simulink model "flightControlSystem"  (R2026b)
settings: Solver=ode3  StopTime=TFinal
PreLoadFcn:
  | InitVars;
undefined symbols (not defined in the file): control_power, feedforward_gains, integrator_limits, MC_PITCH_P, MC_PITCHRATE_D, MC_PITCHRATE_I, MC_PITCHRATE_MAX, MC_PITCHRATE_P, MC_ROLL_P, MC_ROLLRATE_D, MC_ROLLRATE_I, MC_ROLLRATE_MAX, MC_ROLLRATE_P, MC_YAW_P, MC_YAW_TQ_CUTOFF, MC_YAW_WEIGHT, MC_YAWRATE_D, MC_YAWRATE_I, MC_YAWRATE_MAX, MC_YAWRATE_P, MPC_ACC_DECOUPLE, MPC_LAND_ALT1, MPC_LAND_ALT2, MPC_LAND_ALT3, MPC_LAND_CRWL, MPC_LAND_SPEED, MPC_THR_HOVER, MPC_THR_MAX, MPC_THR_MIN, MPC_THR_XY_MARG, MPC_TILTMAX_AIR, MPC_VELD_LP, MPC_XY_P, MPC_XY_VEL_D_ACC, MPC_XY_VEL_I_ACC, MPC_XY_VEL_MAX, MPC_XY_VEL_P_ACC, MPC_Z_P, MPC_Z_VEL_D_ACC, MPC_Z_VEL_I_ACC, MPC_Z_VEL_MAX_DN, MPC_Z_VEL_MAX_UP, MPC_Z_VEL_P_ACC, SampleTime, timestamp
libraries: px4uORBlib x9, vrlib x8, aerolibutil x8, simulink x4, px4Utilslib x4, sharedutil x3, matrix_library x3, raspberrypiutilitieslib x2, px4Peripheralslib x2, sharedtransform x1, px4Sensorslib x1
(part 1 of 4)
settings Model: SimulationMode=external  Creator=The MathWorks, Inc.  LastModifiedBy=merwyn
settings SolverCC: AutoInsertRateTranBlk=on  PositivePriorityOrder=on
settings OptimizationCC: DifferentSizesBufferReuse=on  EfficientTunableParamExpr=on  EnhancedBackFolding=on  MaxStackSize=64  OptimizationCustomize=off  OptimizeBlockOrder=speed  PassReuseOutputArgsAs=Individual arguments  RemoveInternalMemoryZeroInit=on  RemoveRootLevelIOMemoryZeroInit=on
settings DebuggingCC: ParameterPrecisionLossMsg=none  ParameterTunabilityLossMsg=error
settings HardwareCC: ProdHWDeviceType=ARM Compatible->ARM Cortex  ProdLargestAtomicFloat=Double  ProdLargestAtomicInteger=Long  ProdLongLongMode=on
settings SFSimCC: MATLABDynamicMemAlloc=off  SimTargetLang=C++
settings RTWCC: Description=Embedded Coder  GenCodeOnly=on  HardwareBoard=PX4 Pixhawk 6c  SystemTargetFile=ert.tlc  TLCOptions="-aInlineSetEventsForThisBaseRateFcn=TLC_FALSE -aSuppressMultiTaskScheduler=TLC_FALSE  -aRateBasedStepFcn=0"  TargetLang=C++  TemplateMakefile=ert_default_tmf  Toolchain=GNU Tools for PX4 Autopilots
settings CodeAppCC: ForceParamTrailComments=on  IgnoreCustomStorageClasses=off  InsertBlockDesc=on  OperatorAnnotations=on  SFDataObjDesc=on  SimulinkDataObjDesc=on
settings ERTTargetCC: ExtModeIntrfLevel=Level2 - Open  ExtModeMexFile=ext_xcp  ExtModeStaticAlloc=on  SupportContinuousTime=on  SupportVariableSizeSignals=on

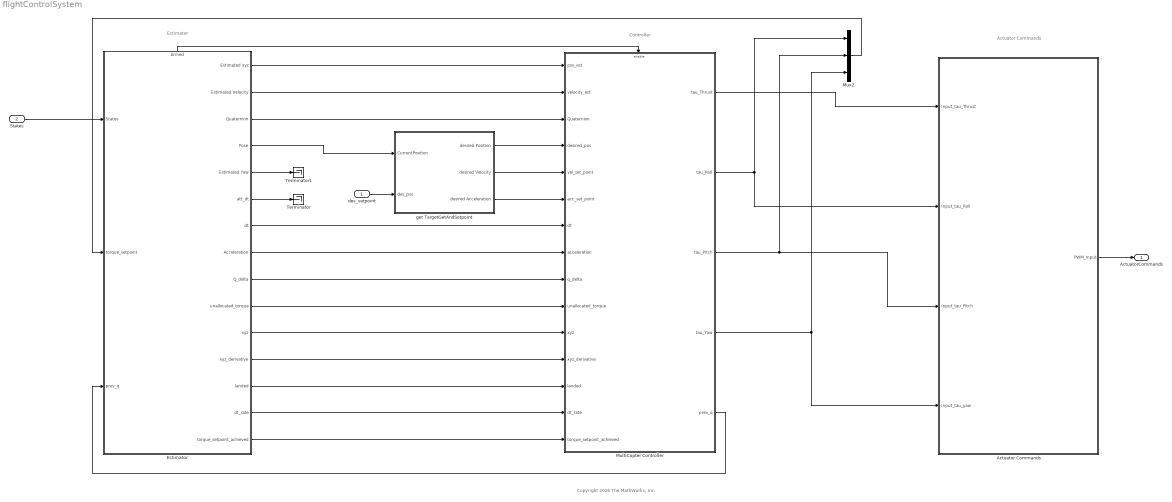
== system flightControlSystem ==
  note: Actuator Commands
  note: Estimator
  note: Controller
  note: Copyright 2026 The MathWorks, Inc.
  des_setpoint : Inport  OutDataTypeStr=Bus: desiredTargetSetpoints
  States : Inport  Port=2  OutDataTypeStr=Bus: UAVStatesBus
  Actuator Commands : Subsystem  Variant=on
  Estimator : Subsystem  Variant=on
      settings: PortSchema="{\"entries\":[{\"content\":{\"sides\":[{\"content\":{\"connectorIds\":[\"In1\",\"In2\",\"In3\"]},\"type\":\"ConnectorPlacement.EquallySpacedRectSide\",\"uuid\":\"982d90d8-ff1f-4cb9-8e33-8baf717922ad\"},{\"content\":{\"connectorIds\":[\"Out1\",\"Out2\",\"Out3\",\"Out4\",\"Out5\",\"Out6\",\"Out7\",\"Out8\",\"Out9\",\"Out10\",\"Out11\",\"Out12\",\"Out13\",\"Out14\",\"Out15\"],\"side\":\"RIGHT\"},\"type\":\"ConnectorPlacement.EquallySpacedRectSide\",\"uuid\":\"20bc02a1-8188-433b-a626-e8822f00966c\"},{\"content\":{\"connectorIds\":[\"Out16\"],\"side\":\"TOP\"},\"type\":\"ConnectorPlacement.EquallySpacedRectSide\",\"uuid\":\"edaeaf83-210e-410d-8d39-7cda3629118d\"}]},\"type\":\"ConnectorPlacement.EquallySpacedConnector\",\"uuid\":\"c0d6638f-6096-4882-ba89-b56950bc4adf\"}],\"packageUris\":[\"http://schema.mathworks.com/mf0/Connector/R2020b\"],\"version\":\"1.0\"}"
  MultiCopter Controller : Subsystem
  Mux2 : Mux  Inputs=3
  Terminator : Terminator
  Terminator1 : Terminator
  get TargetGetAndSetpoint : Subsystem  Variant=on
  ActuatorCommands : Outport  OutDataTypeStr=Bus: setPWMInput
  wires:
  MultiCopter Controller/2(tau_Roll) -> Actuator Commands/2(Input_tau_Roll), Mux2/1
  MultiCopter Controller/1(tau_Thrust) -> Actuator Commands/1(Input_tau_Thrust)
  Estimator/11(xyz) -> MultiCopter Controller/11(xyz)
  MultiCopter Controller/4(tau_Yaw) -> Mux2/3, Actuator Commands/4(Input_tau_yaw)
  Estimator/3(Quaternion) -> MultiCopter Controller/3(Quaternion)
  MultiCopter Controller/5(prev_q) -> Estimator/3(prev_q)
  get TargetGetAndSetpoint/3(desired Acceleration) -> MultiCopter Controller/6(acc_set_point)
  MultiCopter Controller/3(tau_Pitch) -> Actuator Commands/3(Input_tau_Pitch), Mux2/2
  Estimator/10(unallocated_torque) -> MultiCopter Controller/10(unallocated_torque)
  Estimator/12(xyz_derivative) -> MultiCopter Controller/12(xyz_derivative)
  Mux2/1 -> Estimator/2(torque_setpoint)
  Estimator/7(dt) -> MultiCopter Controller/7(dt)
  get TargetGetAndSetpoint/1(desired Position) -> MultiCopter Controller/4(desired_pos)
  Estimator/2(Estimated Velocity) -> MultiCopter Controller/2(velocity_est)
  Estimator/8(Acceleration) -> MultiCopter Controller/8(acceleration)
  Estimator/5(Estimated Yaw) -> Terminator1/1
  Estimator/6(att_dt) -> Terminator/1
  States/1 -> Estimator/1(States)
  Actuator Commands/1(PWM_Input) -> ActuatorCommands/1
  Estimator/13(landed) -> MultiCopter Controller/13(landed)
  get TargetGetAndSetpoint/2(desired Velocity) -> MultiCopter Controller/5(vel_set_point)
  Estimator/4(Pose) -> get TargetGetAndSetpoint/1(CurrentPosition)
  Estimator/1(Estimated xyz) -> MultiCopter Controller/1(pos_est)
  Estimator/9(Q_delta) -> MultiCopter Controller/9(q_delta)
  Estimator/16(Armed) -> MultiCopter Controller/Enable
  Estimator/14(dt_rate) -> MultiCopter Controller/14(dt_rate)
  Estimator/15(torque_setpoint_achieved) -> MultiCopter Controller/15(torque_setpoint_achieved)
  des_setpoint/1 -> get TargetGetAndSetpoint/2(des_pos)

== system flightControlSystem/Actuator Commands ==
  note: Simulation = true:
      | The subsystem processes the tau and thrust signals, computes the multicopter mixers, and generates the PWM signals required by the plant for closed-loop simulation.
      |
      | Simulation = false:
      | The subsystem processes the tau and thrust signals output from the controller and publishes them to the Torque and Thrust block. The PX4 mixer then computes the required outputs based on the selected multicopter configuration for flight operations.
  Input_tau_Thrust : Inport
  Input_tau_Roll : Inport  Port=2
  Input_tau_Pitch : Inport  Port=3
  Input_tau_yaw : Inport  Port=4
  Actuator Commands : Subsystem  VariantControl=Simulation == false
  Simulation Actuator Commands : Subsystem  VariantControl=Simulation == true
  PWM_Input : Outport

== system flightControlSystem/Estimator ==
  note: Simulation = true:
      | The subsystem provides the required estimator values from the 6-DoF Dynamics feedback for closed-loop simulation with the controller.
      |
      | Simulation = false:
      | The subsystem reads the required PX4 estimator values for the flight controller from the uOrb block.
  States : Inport
  torque_setpoint : Inport  Port=2
  prev_q : Inport  Port=3
  Estimator : Subsystem  VariantControl=Simulation == false
  Simulation Estimator : Subsystem  VariantControl=Simulation == true
  Estimated xyz : Outport
  Estimated Velocity : Outport  Port=2
  Quaternion : Outport  Port=3
  Pose : Outport  Port=4
  Estimated Yaw : Outport  Port=5
  att_dt : Outport  Port=6
  dt : Outport  Port=7
  Acceleration : Outport  Port=8
  Q_delta : Outport  Port=9
  unallocated_torque : Outport  Port=10
  xyz : Outport  Port=11
  xyz_derivative : Outport  Port=12
  landed : Outport  Port=13
  dt_rate : Outport  Port=14
  torque_setpoint_achieved : Outport  Port=15
  Armed : Outport  Port=16

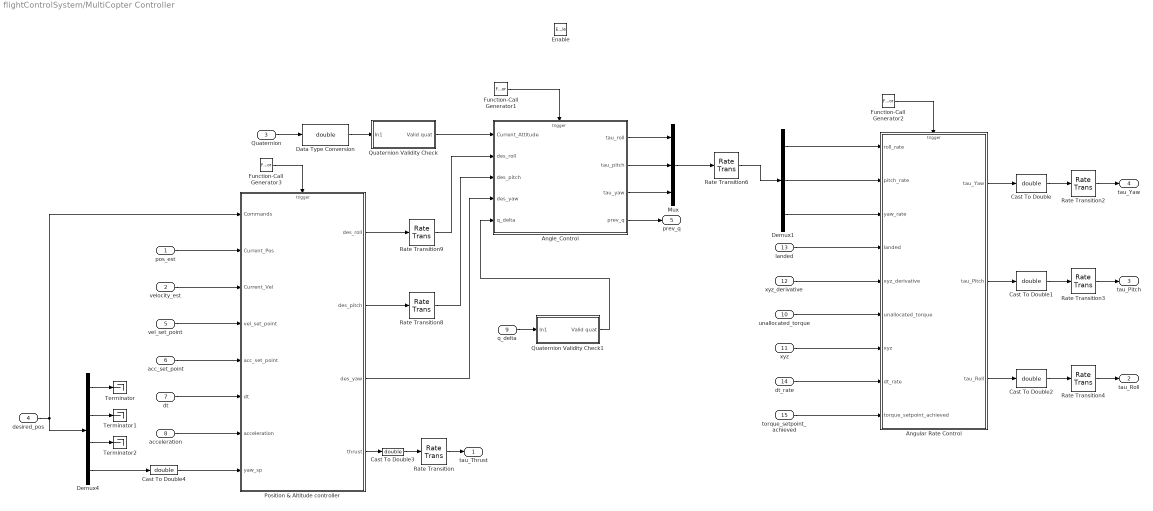
== system flightControlSystem/MultiCopter Controller ==
  pos_est : Inport
  velocity_est : Inport  Port=2
  Quaternion : Inport  Port=3
  desired_pos : Inport  Port=4
  vel_set_point : Inport  Port=5
  acc_set_point : Inport  Port=6
  dt : Inport  Port=7
  acceleration : Inport  Port=8
  q_delta : Inport  Port=9
  unallocated_torque : Inport  Port=10
  xyz : Inport  Port=11
  xyz_derivative : Inport  Port=12
  landed : Inport  Port=13
  dt_rate : Inport  Port=14
  torque_setpoint_achieved : Inport  Port=15
  Enable : EnablePort
  Angle_Control : Subsystem
  Angular Rate Control : Subsystem
  Cast To Double{,1..4} (5 alike) : DataTypeConversion  OutDataTypeStr=double  SaturateOnIntegerOverflow=off  RndMeth=Floor
  Data Type Conversion : DataTypeConversion  OutDataTypeStr=double  SaturateOnIntegerOverflow=off  RndMeth=Floor
  Demux1 : Demux  Outputs=3
  Demux4 : Demux
  Function-Call Generator1 : FunctionCallGenerator  SampleTime=0.004
  Function-Call Generator2 : FunctionCallGenerator  SampleTime=0.001
  Function-Call Generator3 : FunctionCallGenerator  SampleTime=0.02
  Mux : Mux  Inputs=3
  Position & Altitude controller : Subsystem
  Quaternion Validity Check : Subsystem
  Quaternion Validity Check1 : Subsystem
  Rate Transition{,2..4} (4 alike) : RateTransition  OutPortSampleTime=SampleTime
  Rate Transition6 : RateTransition
  Rate Transition8 : RateTransition
  Rate Transition9 : RateTransition
  Terminator : Terminator
  Terminator1 : Terminator
  Terminator2 : Terminator
  tau_Thrust : Outport
  tau_Roll : Outport  Port=2
  tau_Pitch : Outport  Port=3
  tau_Yaw : Outport  Port=4
  prev_q : Outport  Port=5
  wires:
  unallocated_torque/1 -> Angular Rate Control/6(unallocated_torque)
  Demux4/4 -> Cast To Double4/1
  Demux4/2 -> Terminator1/1
  Demux4/3 -> Terminator2/1
  Data Type Conversion/1 -> Quaternion Validity Check/1(In1)
  Quaternion/1 -> Data Type Conversion/1
  Quaternion Validity Check/1(Valid quat) -> Angle_Control/1(Current_Attitude)
  desired_pos/1 -> Position & Altitude controller/1(Commands), Demux4/1
  Demux4/1 -> Terminator/1
  q_delta/1 -> Quaternion Validity Check1/1(In1)
  Function-Call Generator3/1 -> Position & Altitude controller/Trigger
  Angle_Control/4(prev_q) -> prev_q/1
  pos_est/1 -> Position & Altitude controller/2(Current_Pos)
  dt_rate/1 -> Angular Rate Control/8(dt_rate)
  velocity_est/1 -> Position & Altitude controller/3(Current_Vel)
  xyz_derivative/1 -> Angular Rate Control/5(xyz_derivative)
  vel_set_point/1 -> Position & Altitude controller/4(vel_set_point)
  Rate Transition4/1 -> tau_Roll/1
  Angular Rate Control/3("tau_Roll ") -> Cast To Double2/1
  Cast To Double4/1 -> Position & Altitude controller/8(yaw_sp)
  acc_set_point/1 -> Position & Altitude controller/5(acc_set_point)
  dt/1 -> Position & Altitude controller/6(dt)
  Rate Transition2/1 -> tau_Yaw/1
  Quaternion Validity Check1/1(Valid quat) -> Angle_Control/5(q_delta)
  acceleration/1 -> Position & Altitude controller/7(acceleration)
  Position & Altitude controller/2(des_pitch) -> Rate Transition8/1
  Position & Altitude controller/3(des_yaw) -> Angle_Control/4(des_yaw)
  Position & Altitude controller/1(des_roll) -> Rate Transition9/1
  Position & Altitude controller/4(thrust) -> Cast To Double3/1
  Function-Call Generator1/1 -> Angle_Control/Trigger
  Rate Transition9/1 -> Angle_Control/2(des_roll)
  Rate Transition8/1 -> Angle_Control/3(des_pitch)
  Cast To Double3/1 -> Rate Transition/1
  Rate Transition6/1 -> Demux1/1
  landed/1 -> Angular Rate Control/4(landed)
  Rate Transition/1 -> tau_Thrust/1
  Mux/1 -> Rate Transition6/1
  Function-Call Generator2/1 -> Angular Rate Control/Trigger
  Rate Transition3/1 -> tau_Pitch/1
  xyz/1 -> Angular Rate Control/7(xyz)
  torque_setpoint_achieved/1 -> Angular Rate Control/9(torque_setpoint_achieved)
  Angular Rate Control/1(tau_Yaw) -> Cast To Double/1
  Angular Rate Control/2(tau_Pitch) -> Cast To Double1/1
  Cast To Double1/1 -> Rate Transition3/1
  Cast To Double/1 -> Rate Transition2/1
  Cast To Double2/1 -> Rate Transition4/1
  Angle_Control/1(tau_roll) -> Mux/1
  Angle_Control/2(tau_pitch) -> Mux/2
  Angle_Control/3(tau_yaw) -> Mux/3
  Demux1/1 -> Angular Rate Control/1(roll_rate)
  Demux1/2 -> Angular Rate Control/2(pitch_rate)
  Demux1/3 -> Angular Rate Control/3(yaw_rate)

== system flightControlSystem/get TargetGetAndSetpoint ==
  note: Simulation = true:
      | The subsystem forwards the target setpoint signal from the PerceptionGuidance block as a bus signal for controller processing.
      |
      | Simulation = false:
      | The subsystem reads the target setpoint values from the Serial Read block and makes them available to the flight controller.
  CurrentPosition : Inport
  des_pos : Inport  Port=2
  Set target Position : Subsystem  VariantControl=Simulation == false
  Simulation Set target Position : Subsystem  VariantControl=Simulation == true
  desired Position : Outport
  desired Velocity : Outport  Port=2
  desired Acceleration : Outport  Port=3

== system flightControlSystem/Actuator Commands/Actuator Commands ==
  Input_tau_Thrust : Inport
  Input_tau_Pitch : Inport  Port=2
  Input_tau_Roll : Inport  Port=3
  Input_tau_yaw : Inport  Port=4
  Bus Creator1 : BusCreator  Inputs=8  OutDataTypeStr=Bus: setPWMInput
  Demux2 : Demux  Outputs=8
  MATLAB Function : MATLAB Function  TreatAsAtomicUnit=on
  "Using PX4 Mixers " : Subsystem  VariantControl=isUsingSimulinkMixer==false
  PWM_Input : Outport
  wires:
  MATLAB Function/1(y) -> Demux2/1
  Input_tau_Thrust/1 -> "Using PX4 Mixers "/1(tau_Thrust)
  Input_tau_Pitch/1 -> "Using PX4 Mixers "/2(tau_Pitch)
  Input_tau_Roll/1 -> "Using PX4 Mixers "/3(tau_Roll)
  Demux2/7 -> Bus Creator1/7  "M7"
  Demux2/5 -> Bus Creator1/5  "M5"
  Demux2/1 -> Bus Creator1/1  "M1"
  Demux2/3 -> Bus Creator1/3  "M3"
  Demux2/8 -> Bus Creator1/8  "M8"
  Demux2/6 -> Bus Creator1/6  "M6"
  Demux2/4 -> Bus Creator1/4  "M4"
  Demux2/2 -> Bus Creator1/2  "M2"
  Input_tau_yaw/1 -> "Using PX4 Mixers "/4(tau_yaw)
  Bus Creator1/1 -> PWM_Input/1

== system flightControlSystem/Actuator Commands/Simulation Actuator Commands ==
  Input_tau_Thrust : Inport
  Input_tau_Pitch : Inport  Port=2
  Input_tau_Roll : Inport  Port=3
  Input_tau_yaw : Inport  Port=4
  Mixer : Subsystem
  PWM_Input : Outport
  wires:
  Input_tau_Thrust/1 -> Mixer/1(tau_Thrust)
  Mixer/1(PWM_Input) -> PWM_Input/1
  Input_tau_yaw/1 -> Mixer/2(tau_yaw)
  Input_tau_Pitch/1 -> Mixer/3(tau_Pitch)
  Input_tau_Roll/1 -> Mixer/4(tau_Roll)

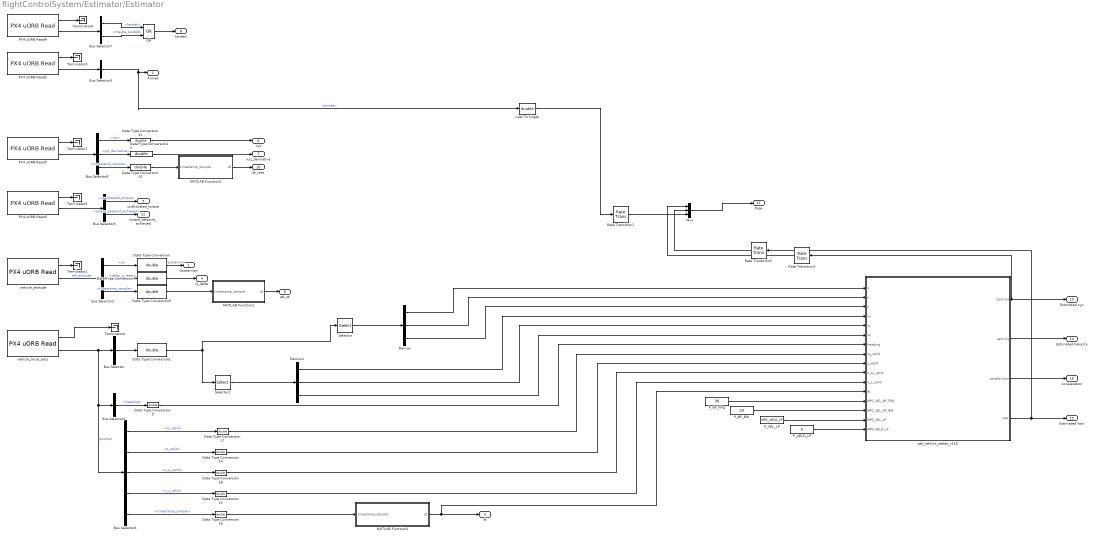
== system flightControlSystem/Estimator/Estimator ==
  Bus Selector : BusSelector  OutputSignals=x,y,z,vx,vy,vz,heading  OutputAsBus=on
  Bus Selector2 : BusSelector  OutputSignals=q,delta_q_reset,timestamp_sample
  Bus Selector3 : BusSelector  OutputSignals=armed
  Bus Selector4 : BusSelector  OutputSignals=heading
  Bus Selector5 : BusSelector  OutputSignals=unallocated_torque,torque_setpoint_achieved
  Bus Selector6 : BusSelector  OutputSignals=xy_valid,z_valid,v_xy_valid,v_z_valid,timestamp_sample
  Bus Selector7 : BusSelector  OutputSignals=landed,maybe_landed
  Bus Selector8 : BusSelector  OutputSignals=xyz,xyz_derivative,timestamp_sample
  Cast To Single : DataTypeConversion  OutDataTypeStr=double  SaturateOnIntegerOverflow=off  RndMeth=Floor
  Data Type Conversion{,1,4..5,9..10,14..18,21..22} (13 alike) : DataTypeConversion  OutDataTypeStr=double  SaturateOnIntegerOverflow=off  RndMeth=Floor
  Demux : Demux  Outputs=3
  Demux1 : Demux  Outputs=3
  MATLAB Function1 : MATLAB Function  TreatAsAtomicUnit=on
  MATLAB Function2 : MATLAB Function  TreatAsAtomicUnit=on
  MATLAB Function4 : MATLAB Function  TreatAsAtomicUnit=on
  Mux : Mux  Inputs=3
  OR : Logic  Operator=OR  IconShape=distinctive  AllPortsSameDT=off  OutDataTypeStr=boolean
  PX4 uORB Read2 : px4uORBlib/PX4 uORB Read  uORBMsg=ActuatorArmed  uORBTopicName=ActuatorArmed  SubscribeNonZeroInstance=off  selectInstanceNum=1  SampleTime=-1  isSingleTopicMsg=off  BlockingMode=off  BlockTimeout=1e-3
  PX4 uORB Read3 : px4uORBlib/PX4 uORB Read  uORBMsg=ControlAllocatorStatus  uORBTopicName=ControlAllocatorStatus  SubscribeNonZeroInstance=off  selectInstanceNum=1  SampleTime=-1  isSingleTopicMsg=off  BlockingMode=off  BlockTimeout=1e-3
  PX4 uORB Read4 : px4uORBlib/PX4 uORB Read  uORBMsg=VehicleLandDetected  uORBTopicName=VehicleLandDetected  SubscribeNonZeroInstance=off  selectInstanceNum=1  SampleTime=-1  isSingleTopicMsg=off  BlockingMode=off  BlockTimeout=1e-3
  PX4 uORB Read5 : px4uORBlib/PX4 uORB Read  uORBMsg=VehicleAngularVelocity  uORBTopicName=vehicle_angular_velocity  SubscribeNonZeroInstance=off  selectInstanceNum=1  SampleTime=-1  isSingleTopicMsg=off  BlockingMode=off  BlockTimeout=1e-3
  P_NF_BW : Constant  Value=20  SampleTime=-1
  P_NF_FRQ : Constant  Value=30  SampleTime=-1
  P_VELD_LP : Constant  Value=5  SampleTime=-1
  P_VEL_LP : Constant  Value=MPC_VELD_LP  SampleTime=-1
  Rate Transition1 : RateTransition
  Rate Transition2 : RateTransition
  Rate Transition3 : RateTransition
  Selector : Selector  InputPortWidth=7  IndexOptions=Index vector (dialog)  Indices=[1:3]  OutputSizes=1  RuntimeRangeChecks=off
  Selector1 : Selector  InputPortWidth=7  IndexOptions=Index vector (dialog)  Indices=[4:6]  OutputSizes=1  RuntimeRangeChecks=off
  Terminator{1,3..7} (6 alike) : Terminator
  set_vehicle_states_v116 : MATLAB Function  TreatAsAtomicUnit=on
  vehicle_attitude : px4uORBlib/PX4 uORB Read  uORBMsg=VehicleAttitude  uORBTopicName=vehicle_attitude  SubscribeNonZeroInstance=off  selectInstanceNum=1  SampleTime=-1  isSingleTopicMsg=off  BlockingMode=off  BlockTimeout=1e-3
  vehicle_local_pos1 : px4uORBlib/PX4 uORB Read  uORBMsg=VehicleLocalPosition  uORBTopicName=vehicle_local_position  SubscribeNonZeroInstance=off  selectInstanceNum=1  SampleTime=-1  isSingleTopicMsg=off  BlockingMode=off  BlockTimeout=1e-3
  "Quaternion " : Outport
  Armed : Outport  Port=2
  dt : Outport  Port=3
  Q_delta : Outport  Port=4
  unallocated_torque : Outport  Port=5
  xyz : Outport  Port=6
  xyz_derivative : Outport  Port=7
  landed : Outport  Port=8
  att_dt : Outport  Port=9
  dt_rate : Outport  Port=10
  torque_setpoint_achieved : Outport  Port=11
  Pose : Outport  Port=12
  Estimated xyz : Outport  Port=13
  Estimated Velocity : Outport  Port=14
  Estimated Yaw : Outport  Port=15
  Acceleration : Outport  Port=16
  wires:
  Data Type Conversion/1 -> "Quaternion "/1  "quaternion"
  PX4 uORB Read2/1 -> Terminator3/1
  PX4 uORB Read3/2 -> Bus Selector5/1
  OR/1 -> landed/1
  PX4 uORB Read4/2 -> Bus Selector7/1
  PX4 uORB Read3/1 -> Terminator5/1
  Data Type Conversion1/1 -> Selector/1, Selector1/1
  PX4 uORB Read2/2 -> Bus Selector3/1
  PX4 uORB Read4/1 -> Terminator6/1
  Data Type Conversion14/1 -> set_vehicle_states_v116/9(z_valid)
  Data Type Conversion10/1 -> MATLAB Function2/1(timestamp_sample)
  PX4 uORB Read5/2 -> Bus Selector8/1
  Selector/1 -> Demux/1
  PX4 uORB Read5/1 -> Terminator7/1
  Data Type Conversion18/1 -> set_vehicle_states_v116/10(v_xy_valid)
  vehicle_attitude/1 -> Terminator1/1
  Data Type Conversion15/1 -> set_vehicle_states_v116/11(v_z_valid)
  vehicle_attitude/2 -> Bus Selector2/1  "ekf_attitude"
  Data Type Conversion22/1 -> xyz_derivative/1
  vehicle_local_pos1/1 -> Terminator4/1
  Data Type Conversion4/1 -> Q_delta/1
  vehicle_local_pos1/2 -> Bus Selector/1, Bus Selector4/1, Bus Selector6/1  "position"
  Bus Selector8/1 -> Data Type Conversion21/1  "<xyz>"
  Bus Selector7/1 -> OR/1  "<landed>"
  Bus Selector8/2 -> Data Type Conversion22/1  "<xyz_derivative>"
  Bus Selector7/2 -> OR/2  "<maybe_landed>"
  Demux1/1 -> set_vehicle_states_v116/4(vx)
  Demux/2 -> set_vehicle_states_v116/2(y)
  Data Type Conversion9/1 -> MATLAB Function1/1(timestamp_sample)
  Bus Selector2/2 -> Data Type Conversion4/1  "<delta_q_reset>"
  Bus Selector3/1 -> Cast To Single/1, Armed/1  "<armed>"
  Bus Selector8/3 -> Data Type Conversion10/1  "<timestamp_sample>"
  Bus Selector6/2 -> Data Type Conversion14/1  "<z_valid>"
  Bus Selector5/1 -> unallocated_torque/1  "<unallocated_torque>"
  Bus Selector6/4 -> Data Type Conversion15/1  "<v_z_valid>"
  Bus Selector5/2 -> torque_setpoint_achieved/1  "<torque_setpoint_achieved>"
  Demux/1 -> set_vehicle_states_v116/1(x)
  Bus Selector4/1 -> Data Type Conversion5/1  "<heading>"
  Bus Selector2/1 -> Data Type Conversion/1  "<q>"
  Demux1/2 -> set_vehicle_states_v116/5(vy)
  Demux/3 -> set_vehicle_states_v116/3(z)
  Bus Selector2/3 -> Data Type Conversion9/1  "<timestamp_sample>"
  Bus Selector/1 -> Data Type Conversion1/1
  Data Type Conversion16/1 -> MATLAB Function4/1(timestamp_sample)
  Data Type Conversion21/1 -> xyz/1
  Data Type Conversion5/1 -> set_vehicle_states_v116/7(heading)
  Bus Selector6/5 -> Data Type Conversion16/1  "<timestamp_sample>"
  Bus Selector6/1 -> Data Type Conversion17/1  "<xy_valid>"
  Bus Selector6/3 -> Data Type Conversion18/1  "<v_xy_valid>"
  MATLAB Function2/1(dt) -> dt_rate/1
  MATLAB Function1/1(dt) -> att_dt/1
  Selector1/1 -> Demux1/1
  Data Type Conversion17/1 -> set_vehicle_states_v116/8(xy_valid)
  Demux1/3 -> set_vehicle_states_v116/6(vz)
  MATLAB Function4/1(dt) -> set_vehicle_states_v116/12(dt), dt/1
  Rate Transition1/1 -> Mux/3
  Mux/1 -> Pose/1
  P_NF_FRQ/1 -> set_vehicle_states_v116/13(MPC_VEL_NF_FRQ)
  P_NF_BW/1 -> set_vehicle_states_v116/14(MPC_VEL_NF_BW)
  P_VEL_LP/1 -> set_vehicle_states_v116/15(MPC_VEL_LP)
  P_VELD_LP/1 -> set_vehicle_states_v116/16(MPC_VELD_LP)
  set_vehicle_states_v116/1(position) -> Estimated xyz/1, Rate Transition3/1
  set_vehicle_states_v116/2(velocity) -> Estimated Velocity/1
  set_vehicle_states_v116/3(acceleration) -> Acceleration/1
  set_vehicle_states_v116/4(yaw) -> Rate Transition2/1, Estimated Yaw/1
  Rate Transition2/1 -> Mux/2
  Rate Transition3/1 -> Mux/1
  Cast To Single/1 -> Rate Transition1/1

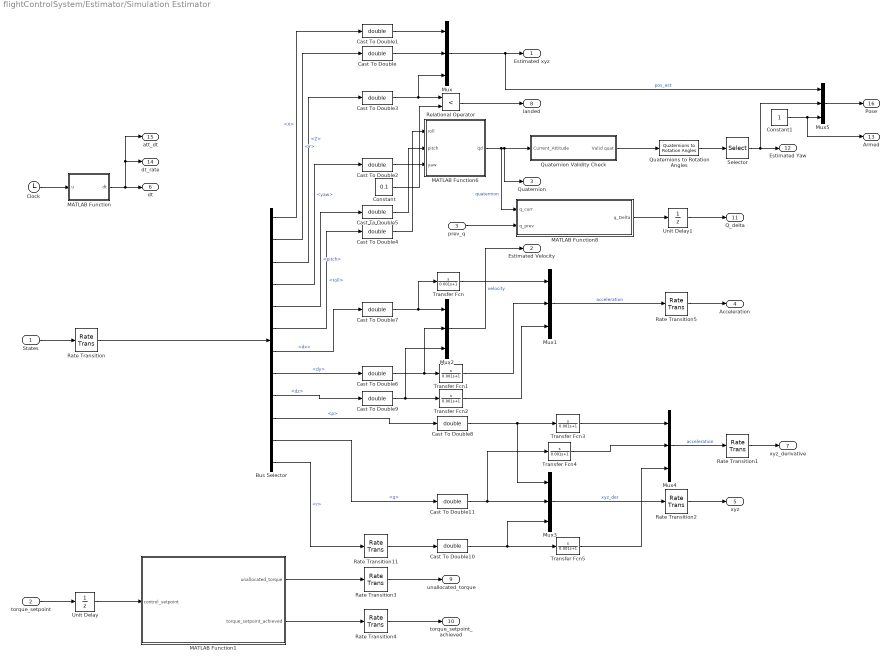
== system flightControlSystem/Estimator/Simulation Estimator ==
  States : Inport
  torque_setpoint : Inport  Port=2
  prev_q : Inport  Port=3
  Bus Selector : BusSelector  OutputSignals=X,Y,Z,yaw,pitch,roll,dx,dy,dz,p,q,r
  Cast To Double{,1..11} (12 alike) : DataTypeConversion  OutDataTypeStr=double  SaturateOnIntegerOverflow=off  RndMeth=Floor
  Clock : Clock
  Constant : Constant  Value=0.1  SampleTime=-1
  Constant1 : Constant  SampleTime=-1
  MATLAB Function : MATLAB Function  TreatAsAtomicUnit=on
  MATLAB Function1 : MATLAB Function  TreatAsAtomicUnit=on
  MATLAB Function6 : MATLAB Function  TreatAsAtomicUnit=on
  MATLAB Function8 : MATLAB Function  TreatAsAtomicUnit=on
  Mux{,1..5} (6 alike) : Mux  Inputs=3
  Quaternion Validity Check : Subsystem
  Quaternions to Rotation Angles : sharedtransform/Quaternions to Rotation Angles  rotationOrder=ZYX  aMode=aMode
  Rate Transition : RateTransition  OutPortSampleTime=SampleTime
  Rate Transition{1..5} (5 alike) : RateTransition
  Rate Transition11 : RateTransition  OutPortSampleTime=SampleTime
  Relational Operator : RelationalOperator  Operator=<  OutDataTypeStr=boolean  RndMeth=Simplest  InputSameDT=off
  Selector : Selector  InputPortWidth=3  IndexOptions=Index vector (dialog)  Indices=1  OutputSizes=1  RuntimeRangeChecks=off
  Transfer Fcn{,1..5} (6 alike) : TransferFcn  Numerator=[1 0]  Denominator=[0.001 1]
  Unit Delay : UnitDelay  InitialCondition=[0,0,0]  SampleTime=-1
  Unit Delay1 : UnitDelay  InitialCondition=[1,0,0,0]  SampleTime=-1
  Estimated xyz : Outport
  Estimated Velocity : Outport  Port=2
  "Quaternion " : Outport  Port=3
  Acceleration : Outport  Port=4
  xyz : Outport  Port=5
  dt : Outport  Port=6
  xyz_derivative : Outport  Port=7
  landed : Outport  Port=8
  unallocated_torque : Outport  Port=9
  torque_setpoint_achieved : Outport  Port=10
  Q_delta : Outport  Port=11
  Estimated Yaw : Outport  Port=12
  Armed : Outport  Port=13
  dt_rate : Outport  Port=14
  att_dt : Outport  Port=15
  Pose : Outport  Port=16
  wires:
  Quaternions to Rotation Angles/1 -> Selector/1
  States/1 -> Rate Transition/1
  Cast To Double1/1 -> Mux/1
  Clock/1 -> MATLAB Function/1(u)
  Selector/1 -> Mux5/2, Estimated Yaw/1
  Constant1/1 -> Mux5/3, Armed/1
  Rate Transition1/1 -> xyz_derivative/1
  Transfer Fcn/1 -> Mux1/1
  torque_setpoint/1 -> Unit Delay/1
  Cast To Double2/1 -> MATLAB Function6/3(yaw)
  Unit Delay/1 -> MATLAB Function1/1(control_setpoint)
  Cast To Double/1 -> Mux/2
  Rate Transition/1 -> Bus Selector/1
  Rate Transition3/1 -> unallocated_torque/1
  Bus Selector/11 -> Cast To Double11/1  "<q>"
  MATLAB Function/1(dt) -> dt_rate/1, att_dt/1, dt/1
  Cast To Double4/1 -> MATLAB Function6/1(roll)
  Bus Selector/1 -> Cast To Double1/1  "<X>"
  Transfer Fcn4/1 -> Mux4/2
  Bus Selector/2 -> Cast To Double/1  "<Y>"
  Bus Selector/3 -> Cast To Double3/1  "<Z>"
  Cast To Double5/1 -> MATLAB Function6/2(pitch)
  Bus Selector/4 -> Cast To Double2/1  "<yaw>"
  Transfer Fcn3/1 -> Mux4/1
  Bus Selector/5 -> Cast To Double5/1  "<pitch>"
  Rate Transition2/1 -> xyz/1
  Bus Selector/6 -> Cast To Double4/1  "<roll>"
  Cast To Double6/1 -> Mux2/2, Transfer Fcn1/1
  Bus Selector/7 -> Cast To Double7/1  "<dx>"
  Transfer Fcn5/1 -> Mux4/3
  Rate Transition4/1 -> torque_setpoint_achieved/1
  Bus Selector/8 -> Cast To Double6/1  "<dy>"
  Rate Transition11/1 -> Cast To Double10/1
  Bus Selector/9 -> Cast To Double9/1  "<dz>"
  Cast To Double7/1 -> Transfer Fcn/1, Mux2/1
  Bus Selector/10 -> Cast To Double8/1  "<p>"
  Bus Selector/12 -> Rate Transition11/1  "<r>"
  MATLAB Function1/1(unallocated_torque) -> Rate Transition3/1
  MATLAB Function1/2(torque_setpoint_achieved) -> Rate Transition4/1
  prev_q/1 -> MATLAB Function8/2(q_prev)
  Cast To Double3/1 -> Relational Operator/1, Mux/3
  Constant/1 -> Relational Operator/2
  Cast To Double9/1 -> Transfer Fcn2/1, Mux2/3
  Mux/1 -> Mux5/1, Estimated xyz/1  "pos_est"
  Transfer Fcn1/1 -> Mux1/2
  Relational Operator/1 -> landed/1
  MATLAB Function6/1(qd) -> "Quaternion "/1, Quaternion Validity Check/1(Current_Attitude), MATLAB Function8/1(q_curr)  "quaternion"
  Mux2/1 -> Estimated Velocity/1  "velocity"
  Transfer Fcn2/1 -> Mux1/3
  Cast To Double8/1 -> Transfer Fcn3/1, Mux3/1
  Unit Delay1/1 -> Q_delta/1
  Cast To Double11/1 -> Transfer Fcn4/1, Mux3/2
  Rate Transition5/1 -> Acceleration/1
  Cast To Double10/1 -> Transfer Fcn5/1, Mux3/3
  Quaternion Validity Check/1(Valid quat) -> Quaternions to Rotation Angles/1
  Mux1/1 -> Rate Transition5/1  "acceleration"
  MATLAB Function8/1(q_Delta) -> Unit Delay1/1
  Mux3/1 -> Rate Transition2/1  "xyz_der"
  Mux4/1 -> Rate Transition1/1  "acceleration"
  Mux5/1 -> Pose/1

== system flightControlSystem/MultiCopter Controller/Angle_Control ==
  Current_Attitude : Inport
  des_roll : Inport  Port=2
  des_pitch : Inport  Port=3
  des_yaw : Inport  Port=4
  q_delta : Inport  Port=5
  function : TriggerPort  TriggerType=function-call  VariantControl=(inherit)
  AttitudeControl : Subsystem
  Cast To Single{,1..7} (8 alike) : DataTypeConversion  OutDataTypeStr=single  SaturateOnIntegerOverflow=off  RndMeth=Floor
  Constant : Constant  Value=[MC_ROLL_P, MC_PITCH_P, MC_YAW_P]  SampleTime=-1
  Constant1 : Constant  Value=MC_YAW_WEIGHT  SampleTime=-1
  Constant3 : Constant  Value=0  SampleTime=-1
  Demux3 : Demux  Outputs=3
  MATLAB Function4 : MATLAB Function  TreatAsAtomicUnit=on
  tau_roll : Outport
  tau_pitch : Outport  Port=2
  tau_yaw : Outport  Port=3
  prev_q : Outport  Port=4
  wires:
  MATLAB Function4/1(qd) -> Cast To Single7/1
  Constant1/1 -> Cast To Single4/1
  Constant3/1 -> Cast To Single5/1
  Current_Attitude/1 -> AttitudeControl/1(q)
  Cast To Single3/1 -> AttitudeControl/4(pGain)
  Cast To Single6/1 -> AttitudeControl/2(qDelta)
  Cast To Single7/1 -> AttitudeControl/3(att_sp_q)
  Cast To Single5/1 -> AttitudeControl/6(yawSpSetpoint)
  Cast To Single4/1 -> AttitudeControl/5(yawWeight)
  AttitudeControl/1(rate_setpoint) -> Demux3/1
  Cast To Single2/1 -> tau_roll/1
  Cast To Single/1 -> tau_yaw/1
  Cast To Single1/1 -> tau_pitch/1
  des_pitch/1 -> MATLAB Function4/2(pitch)  "des_pitch"
  AttitudeControl/2(prev_q) -> prev_q/1
  Demux3/1 -> Cast To Single2/1
  Demux3/2 -> Cast To Single1/1
  Demux3/3 -> Cast To Single/1
  Constant/1 -> Cast To Single3/1
  q_delta/1 -> Cast To Single6/1
  des_yaw/1 -> MATLAB Function4/3(yaw)  "des_yaw"
  des_roll/1 -> MATLAB Function4/1(roll)  "des_roll"

== system flightControlSystem/MultiCopter Controller/Angular Rate Control ==
  roll_rate : Inport
  pitch_rate : Inport  Port=2
  yaw_rate : Inport  Port=3
  landed : Inport  Port=4
  xyz_derivative : Inport  Port=5
  unallocated_torque : Inport  Port=6
  xyz : Inport  Port=7
  dt_rate : Inport  Port=8
  torque_setpoint_achieved : Inport  Port=9
  function : TriggerPort  TriggerType=function-call  VariantControl=(inherit)
  Cast To Double : DataTypeConversion  OutDataTypeStr=double  SaturateOnIntegerOverflow=off  RndMeth=Floor
  Cast To Single : DataTypeConversion  OutDataTypeStr=single  SaturateOnIntegerOverflow=off  RndMeth=Floor
  Constant1 : Constant  Value=integrator_limits  SampleTime=-1
  Constant2 : Constant  Value=feedforward_gains  SampleTime=-1
  Constant3 : Constant  Value=[MC_ROLLRATE_P, MC_PITCHRATE_P, MC_YAWRATE_P]  SampleTime=-1
  Constant4 : Constant  Value=[MC_ROLLRATE_I, MC_PITCHRATE_I, MC_YAWRATE_I]  SampleTime=-1
  Constant5 : Constant  Value=[MC_ROLLRATE_D, MC_PITCHRATE_D, MC_YAWRATE_D]  SampleTime=-1
  Demux : Demux  Outputs=3
  MATLAB Function : MATLAB Function  TreatAsAtomicUnit=on
  Mux : Mux  Inputs=3
  Subsystem : Subsystem
  Unit Delay : UnitDelay  InitialCondition=[0,0,0]  SampleTime=-1
  get TargetGetAndSetpoint : Subsystem  Variant=on
  tau_Yaw : Outport
  tau_Pitch : Outport  Port=2
  "tau_Roll " : Outport  Port=3
  wires:
  yaw_rate/1 -> Mux/3  "yaw_rate"
  MATLAB Function/1(control_power) -> Cast To Single/1
  dt_rate/1 -> Cast To Double/1
  roll_rate/1 -> Mux/1  "roll_rate"
  pitch_rate/1 -> Mux/2  "pitch_rate"
  xyz/1 -> Subsystem/1(rate)
  Constant5/1 -> Subsystem/8(D)
  Mux/1 -> Subsystem/2(rate_sp)
  torque_setpoint_achieved/1 -> Subsystem/3(torque_setpoint_achieved)
  landed/1 -> Subsystem/4(landed)
  unallocated_torque/1 -> Subsystem/5(unallocated_torque)
  Constant3/1 -> Subsystem/6(P)
  Constant4/1 -> Subsystem/7(I)
  Constant1/1 -> Subsystem/9(lim_int)
  xyz_derivative/1 -> Subsystem/11(angular_accel)
  Constant2/1 -> Subsystem/12(ff)
  Unit Delay/1 -> Subsystem/13(rate_int_in)
  Cast To Double/1 -> MATLAB Function/2(dt), Subsystem/10(dt)
  Demux/3 -> tau_Yaw/1
  Subsystem/2(rate_int) -> Unit Delay/1
  Subsystem/1(rate_setpoint) -> Demux/1, MATLAB Function/1(vehicle_torque_setpoint)
  Demux/1 -> "tau_Roll "/1
  Demux/2 -> tau_Pitch/1
  Cast To Single/1 -> get TargetGetAndSetpoint/1(Control_Power)

== system flightControlSystem/MultiCopter Controller/Position & Altitude controller ==
  Commands : Inport
  Current_Pos : Inport  Port=2
  Current_Vel : Inport  Port=3
  vel_set_point : Inport  Port=4
  acc_set_point : Inport  Port=5
  dt : Inport  Port=6
  acceleration : Inport  Port=7
  yaw_sp : Inport  Port=8
  function : TriggerPort  TriggerType=function-call  VariantControl=(inherit)
  Cast To Double : DataTypeConversion  OutDataTypeStr=double  SaturateOnIntegerOverflow=off  RndMeth=Floor
  Cast To Double1 : DataTypeConversion  OutDataTypeStr=double  SaturateOnIntegerOverflow=off  RndMeth=Floor
  Cast To Double2 : DataTypeConversion  OutDataTypeStr=double  SaturateOnIntegerOverflow=off  RndMeth=Floor
  Position controller : Subsystem
  Terminator3 : Terminator
  des_roll : Outport
  des_pitch : Outport  Port=2
  des_yaw : Outport  Port=3
  thrust : Outport  Port=4
  wires:
  Current_Vel/1 -> Cast To Double1/1
  Commands/1 -> Position controller/1(Commands)
  Current_Pos/1 -> Cast To Double/1
  acceleration/1 -> Cast To Double2/1
  Cast To Double/1 -> Position controller/2(Current_Pos)
  Cast To Double1/1 -> Position controller/3(Current_Vel)
  Position controller/4(thrust) -> thrust/1
  Position controller/3(roll) -> des_roll/1
  Position controller/2(pitch) -> des_pitch/1
  Position controller/1(yaw) -> des_yaw/1
  dt/1 -> Position controller/7(dt)
  Cast To Double2/1 -> Position controller/8(acceleration)
  yaw_sp/1 -> Position controller/4(yaw_sp)
  vel_set_point/1 -> Position controller/5(velocity_input)
  acc_set_point/1 -> Position controller/6(acc_input)
  Position controller/5(hover_thrust_estimate) -> Terminator3/1

== system flightControlSystem/MultiCopter Controller/Quaternion Validity Check ==
  In1 : Inport
  Constant : Constant  Value=[1 0 0 0]  SampleTime=-1
  Quaternion Norm : sharedutil/Quaternion Norm  aMode=aMode
  Switch : Switch  Criteria=u2 > Threshold  SaturateOnIntegerOverflow=off  InputSameDT=off
  Valid quat : Outport
  wires:
  In1/1 -> Quaternion Norm/1, Switch/1
  Quaternion Norm/1 -> Switch/2
  Switch/1 -> Valid quat/1
  Constant/1 -> Switch/3

== system flightControlSystem/MultiCopter Controller/Quaternion Validity Check1 ==
  In1 : Inport
  Constant : Constant  Value=[1 0 0 0]  SampleTime=-1
  Quaternion Norm : sharedutil/Quaternion Norm  aMode=aMode
  Switch : Switch  Criteria=u2 > Threshold  SaturateOnIntegerOverflow=off  InputSameDT=off
  Valid quat : Outport
  wires:
  In1/1 -> Quaternion Norm/1, Switch/1
  Quaternion Norm/1 -> Switch/2
  Switch/1 -> Valid quat/1
  Constant/1 -> Switch/3

== system flightControlSystem/get TargetGetAndSetpoint/Set target Position ==
  CurrentPosition : Inport
  Landing Logic : Subsystem
  Logger : Subsystem
  RC Failsafe Signal : Subsystem
  Rate Transition1 : RateTransition  OutPortSampleTime=1/10
  Setpoints Selector : Subsystem
  Setpoints from Perception Module : Subsystem
  desired Velocity : Outport
  desired Acceleration : Outport  Port=2
  desired Position : Outport  Port=3
  wires:
  Setpoints Selector/3(des_acc) -> desired Acceleration/1, Logger/3(DesiredAcceleration)
  RC Failsafe Signal/1(Land_Trigger) -> Setpoints Selector/4(LandTrigger), Landing Logic/2(land_trigger)
  CurrentPosition/1 -> Rate Transition1/1
  Landing Logic/1(pos_sp) -> Setpoints Selector/1(Land_Pos)
  Landing Logic/3(acc_sp) -> Setpoints Selector/3(Land_Acc)
  Setpoints Selector/1(des_pos) -> Logger/1(DesiredPosition), desired Position/1
  Setpoints Selector/2(des_vel) -> Logger/2(DesiredVelocity), desired Velocity/1
  Landing Logic/2(vel_sp) -> Setpoints Selector/2(Land_Vel)
  Rate Transition1/1 -> Logger/4(States), Setpoints from Perception Module/1(CurrentPosition), Landing Logic/1(Current_Pos)
  Setpoints from Perception Module/1(des Position) -> Setpoints Selector/5(Des_Pos)
  Setpoints from Perception Module/2(desired Velocity) -> Setpoints Selector/6(Des_Vel)
  Setpoints from Perception Module/3(desired Acceleration) -> Setpoints Selector/7(Des_Acc)

== system flightControlSystem/get TargetGetAndSetpoint/Simulation Set target Position ==
  des_pos : Inport
  CurrentPosition : Inport  Port=2
  Bus to Vector : BusToVector
  Constant : Constant  Value=0  SampleTime=-1
  Constant1 : Constant  SampleTime=-1
  Constant2 : Constant  Value=0  SampleTime=-1
  Demux : Demux  Outputs=11
  Landing Logic : Subsystem
  Mux : Mux
  Mux1 : Mux  Inputs=3
  Mux2 : Mux  Inputs=3
  Setpoints Selector : Subsystem
  Switch1 : Switch  Criteria=u2 ~= 0  SaturateOnIntegerOverflow=off  InputSameDT=off
  Terminator3 : Terminator
  desired Position : Outport
  desired Velocity : Outport  Port=2
  desired Acceleration : Outport  Port=3
  wires:
  Bus to Vector/1 -> Demux/1
  Constant2/1 -> Switch1/2
  des_pos/1 -> Bus to Vector/1
  Constant1/1 -> Switch1/1
  Constant/1 -> Switch1/3
  Switch1/1 -> Setpoints Selector/4(LandTrigger), Landing Logic/2(land_trigger)
  Demux/1 -> Mux/1
  Demux/2 -> Mux/2
  Demux/3 -> Mux/3
  Demux/4 -> Mux/4
  Demux/5 -> Mux1/1
  Demux/6 -> Mux1/2
  Demux/7 -> Mux1/3
  Demux/8 -> Mux2/1
  Demux/9 -> Mux2/2
  Demux/10 -> Mux2/3
  Demux/11 -> Terminator3/1
  Setpoints Selector/1(des_pos) -> desired Position/1
  CurrentPosition/1 -> Landing Logic/1(Current_Pos)
  Landing Logic/1(pos_sp) -> Setpoints Selector/1(Land_Pos)
  Landing Logic/2(vel_sp) -> Setpoints Selector/2(Land_Vel)
  Landing Logic/3(acc_sp) -> Setpoints Selector/3(Land_Acc)
  Mux/1 -> Setpoints Selector/5(Des_Pos)
  Mux1/1 -> Setpoints Selector/6(Des_Vel)
  Mux2/1 -> Setpoints Selector/7(Des_Acc)
  Setpoints Selector/2(des_vel) -> desired Velocity/1
  Setpoints Selector/3(des_acc) -> desired Acceleration/1

== system flightControlSystem/Actuator Commands/Actuator Commands/Using PX4 Mixers  ==
  note: Note:
      | 1. All the values are in the drone body FRD frame.
      | 2. Positive z is downwards in the FRD frame, so 'thrust_z' is negative.
  tau_Thrust : Inport
  tau_Pitch : Inport  Port=2
  tau_Roll : Inport  Port=3
  tau_yaw : Inport  Port=4
  Bus Selector : BusSelector  OutputSignals=voltage_v,current_a,current_average_a,discharged_mah,scale
  Cast To Single{2..5} (4 alike) : DataTypeConversion  OutDataTypeStr=single  SaturateOnIntegerOverflow=off  RndMeth=Floor
  Compare To Constant : simulink/Logic and Bit Operations/Compare To Constant  relop=~=  const=0  OutDataTypeStr=boolean
  PX4 ULog : px4Utilslib/PX4 ULog  Commented=on  uORBMsg=BatteryLogging
  PX4 Write Thrust & Torque Setpoint : px4Utilslib/PX4 Write Thrust & Torque Setpoint
  PX4 uORB Read5 : px4uORBlib/PX4 uORB Read  uORBMsg=BatteryStatus  uORBTopicName=BatteryStatus  SubscribeNonZeroInstance=off  selectInstanceNum=1  SampleTime=-1  isSingleTopicMsg=off  BlockingMode=off  BlockTimeout=1e-3
  Product : Product
  Product1 : Product
  Saturation : Saturate  UpperLimit=1  LowerLimit=-1
  Saturation1 : Saturate  UpperLimit=1  LowerLimit=-1
  Switch : Switch  Criteria=u2 > Threshold  SaturateOnIntegerOverflow=off  InputSameDT=off
  Switch1 : Switch  Criteria=u2 > Threshold  SaturateOnIntegerOverflow=off  InputSameDT=off
  Terminator7 : Terminator
  Vector Concatenate1 : Concatenate  NumInputs=3
  wires:
  PX4 uORB Read5/1 -> Terminator7/1
  PX4 uORB Read5/2 -> Bus Selector/1
  Bus Selector/2 -> Cast To Single3/1  "<current_a>"
  tau_yaw/1 -> Vector Concatenate1/3
  tau_Roll/1 -> Vector Concatenate1/1
  tau_Pitch/1 -> Vector Concatenate1/2
  Bus Selector/1 -> Cast To Single2/1  "<voltage_v>"
  Vector Concatenate1/1 -> Switch1/3, Product1/1
  Bus Selector/3 -> Cast To Single4/1  "<current_average_a>"
  Bus Selector/4 -> Cast To Single5/1  "<discharged_mah>"
  Bus Selector/5 -> Compare To Constant/1, Product/2, Product1/2  "<scale>"
  tau_Thrust/1 -> Switch/3, Product/1
  Cast To Single2/1 -> PX4 ULog/1
  Cast To Single3/1 -> PX4 ULog/2
  Cast To Single4/1 -> PX4 ULog/3
  Cast To Single5/1 -> PX4 ULog/4
  Compare To Constant/1 -> Switch1/2, Switch/2
  Product/1 -> Switch/1
  Product1/1 -> Switch1/1
  Switch/1 -> Saturation1/1
  Switch1/1 -> Saturation/1
  Saturation1/1 -> PX4 Write Thrust & Torque Setpoint/1
  Saturation/1 -> PX4 Write Thrust & Torque Setpoint/2

== system flightControlSystem/Actuator Commands/Simulation Actuator Commands/Mixer ==
  tau_Thrust : Inport
  tau_yaw : Inport  Port=2
  tau_Pitch : Inport  Port=3
  tau_Roll : Inport  Port=4
  Battery_Scaling : Subsystem
  Bus Creator1 : BusCreator  Inputs=8  OutDataTypeStr=Bus: setPWMInput
  Demux : Demux  Outputs=3
  Demux2 : Demux  Outputs=8
  MATLAB Function : MATLAB Function  TreatAsAtomicUnit=on
  Saturation : Saturate  UpperLimit=1  LowerLimit=0
  String Constant : StringConstant  String=frameType
  Terminator : Terminator
  Terminator1 : Terminator
  Vector Concatenate1 : Concatenate  NumInputs=3
  PWM_Input : Outport
  wires:
  Demux/1 -> Terminator/1
  Demux/2 -> Terminator1/1
  Demux/3 -> Battery_Scaling/1(In1)
  tau_Thrust/1 -> Demux/1
  tau_yaw/1 -> Vector Concatenate1/3
  Vector Concatenate1/1 -> Battery_Scaling/2(In2)
  tau_Roll/1 -> Vector Concatenate1/1
  tau_Pitch/1 -> Vector Concatenate1/2
  String Constant/1 -> MATLAB Function/1(frameType)
  Battery_Scaling/4(yaw) -> MATLAB Function/5(yaw)
  Battery_Scaling/3(roll) -> MATLAB Function/4(roll)
  Battery_Scaling/2(pitch) -> MATLAB Function/3(pitch)
  Battery_Scaling/1(thrust_setpoint) -> MATLAB Function/2(thrust)
  Demux2/3 -> Bus Creator1/3  "M3"
  MATLAB Function/1(rotor_cmd) -> Saturation/1
  Demux2/8 -> Bus Creator1/8  "M8"
  Demux2/1 -> Bus Creator1/1  "M1"
  Demux2/2 -> Bus Creator1/2  "M2"
  Demux2/4 -> Bus Creator1/4  "M4"
  Demux2/5 -> Bus Creator1/5  "M5"
  Demux2/6 -> Bus Creator1/6  "M6"
  Demux2/7 -> Bus Creator1/7  "M7"
  Bus Creator1/1 -> PWM_Input/1
  Saturation/1 -> Demux2/1

== system flightControlSystem/Estimator/Simulation Estimator/Quaternion Validity Check ==
  Current_Attitude : Inport
  Constant : Constant  Value=[1 0 0 0]  SampleTime=-1
  Quaternion Norm : sharedutil/Quaternion Norm  aMode=aMode
  Switch : Switch  Criteria=u2 > Threshold  SaturateOnIntegerOverflow=off  InputSameDT=off
  Valid quat : Outport
  wires:
  Current_Attitude/1 -> Quaternion Norm/1, Switch/1
  Quaternion Norm/1 -> Switch/2
  Switch/1 -> Valid quat/1
  Constant/1 -> Switch/3

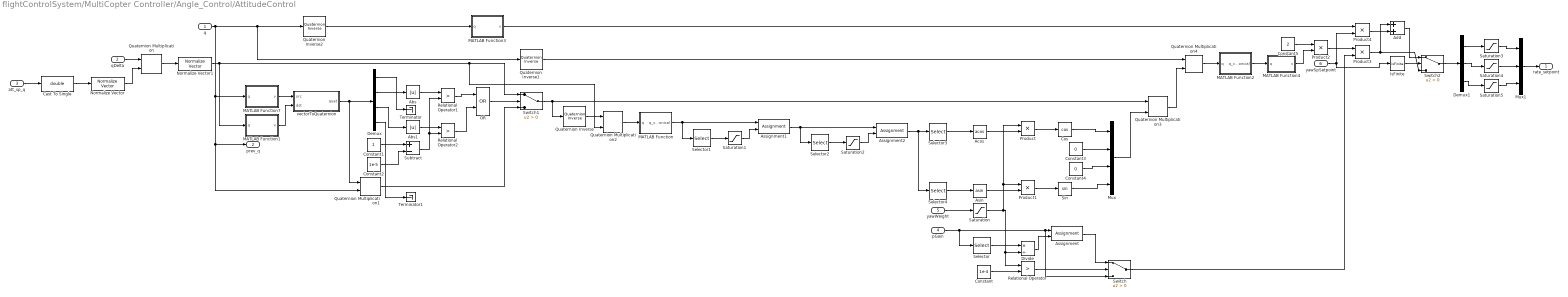
== system flightControlSystem/MultiCopter Controller/Angle_Control/AttitudeControl ==
  q : Inport
  qDelta : Inport  Port=2
  att_sp_q : Inport  Port=3
  pGain : Inport  Port=4
  yawWeight : Inport  Port=5
  yawSpSetpoint : Inport  Port=6
  Abs : Abs  SaturateOnIntegerOverflow=off
  Abs1 : Abs  SaturateOnIntegerOverflow=off
  Acos : Trigonometry  Operator=acos
  Add : Sum
  Asin : Trigonometry  Operator=asin
  Assignment : Assignment  DiagnosticForDimensions=Warning  IndexOptions=Index vector (dialog)  Indices=3  OutputSizes=1  RuntimeRangeChecks=off
  Assignment1 : Assignment  DiagnosticForDimensions=Warning  IndexOptions=Index vector (dialog)  Indices=[1]  OutputSizes=1  RuntimeRangeChecks=off
  Assignment2 : Assignment  DiagnosticForDimensions=Warning  IndexOptions=Index vector (dialog)  Indices=[4]  OutputSizes=1  RuntimeRangeChecks=off
  Cast To Single : DataTypeConversion  OutDataTypeStr=double  SaturateOnIntegerOverflow=off  RndMeth=Floor
  Constant : Constant  Value=1e-4  OutDataTypeStr=single  SampleTime=-1
  Constant1 : Constant  SampleTime=-1
  Constant2 : Constant  Value=1e-5  SampleTime=-1
  Constant3 : Constant  Value=0  OutDataTypeStr=single  SampleTime=-1
  Constant4 : Constant  Value=0  OutDataTypeStr=single  SampleTime=-1
  Constant5 : Constant  Value=2  SampleTime=-1
  Cos : Trigonometry  Operator=cos
  Demux : Demux
  Demux1 : Demux  Outputs=3
  Divide : Product  Inputs=*/
  IsFinite : RelationalOperator  Operator=isFinite  OutDataTypeStr=boolean  RndMeth=Simplest  InputSameDT=off
  MATLAB Function : MATLAB Function  TreatAsAtomicUnit=on
  MATLAB Function1 : MATLAB Function  TreatAsAtomicUnit=on
  MATLAB Function2 : MATLAB Function  TreatAsAtomicUnit=on
  MATLAB Function3 : MATLAB Function  TreatAsAtomicUnit=on
  MATLAB Function4 : MATLAB Function  TreatAsAtomicUnit=on
  MATLAB Function7 : MATLAB Function  TreatAsAtomicUnit=on
  Mux : Mux
  Mux1 : Mux  Inputs=3
  Normalize Vector : vrlib/Utilities/Normalize Vector  maxzero=0
  Normalize Vector1 : vrlib/Utilities/Normalize Vector  maxzero=0
  OR : Logic  Operator=OR  IconShape=distinctive  AllPortsSameDT=off  OutDataTypeStr=boolean
  Product{,1..4} (5 alike) : Product
  Quaternion Inverse : aerolibutil/Quaternion Inverse
  Quaternion Inverse1 : aerolibutil/Quaternion Inverse
  Quaternion Inverse2 : aerolibutil/Quaternion Inverse
  Quaternion Multiplication{,1..4} (5 alike) : aerolibutil/Quaternion Multiplication
  Relational Operator : RelationalOperator  Operator=>  OutDataTypeStr=boolean  RndMeth=Simplest  InputSameDT=off
  Relational Operator1 : RelationalOperator  Operator=>  OutDataTypeStr=boolean  RndMeth=Simplest  InputSameDT=off
  Relational Operator2 : RelationalOperator  Operator=>  OutDataTypeStr=boolean  RndMeth=Simplest  InputSameDT=off
  Saturation : Saturate  UpperLimit=1  LowerLimit=0
  Saturation1 : Saturate  UpperLimit=1  LowerLimit=-1
  Saturation2 : Saturate  UpperLimit=1  LowerLimit=-1
  Saturation3 : Saturate  UpperLimit=deg2rad(MC_ROLLRATE_MAX)  LowerLimit=-deg2rad(MC_ROLLRATE_MAX)
  Saturation4 : Saturate  UpperLimit=deg2rad(MC_PITCHRATE_MAX)  LowerLimit=-deg2rad(MC_PITCHRATE_MAX)
  Saturation5 : Saturate  UpperLimit=deg2rad(MC_YAWRATE_MAX)  LowerLimit=-deg2rad(MC_YAWRATE_MAX)
  Selector : Selector  InputPortWidth=3  IndexOptions=Index vector (dialog)  Indices=[3]  OutputSizes=1  RuntimeRangeChecks=off
  Selector1 : Selector  InputPortWidth=4  IndexOptions=Index vector (dialog)  Indices=[1]  OutputSizes=1  RuntimeRangeChecks=off
  Selector2 : Selector  InputPortWidth=4  IndexOptions=Index vector (dialog)  Indices=[4]  OutputSizes=1  RuntimeRangeChecks=off
  Selector3 : Selector  InputPortWidth=4  IndexOptions=Index vector (dialog)  Indices=[1]  OutputSizes=1  RuntimeRangeChecks=off
  Selector4 : Selector  InputPortWidth=4  IndexOptions=Index vector (dialog)  Indices=[4]  OutputSizes=1  RuntimeRangeChecks=off
  Sin : Trigonometry
  Subtract : Sum  Inputs=+-
  Switch : Switch  Criteria=u2 > Threshold  SaturateOnIntegerOverflow=off  InputSameDT=off
  Switch1 : Switch  Criteria=u2 > Threshold  SaturateOnIntegerOverflow=off  InputSameDT=off
  Switch2 : Switch  Criteria=u2 > Threshold  SaturateOnIntegerOverflow=off  InputSameDT=off
  Terminator : Terminator
  Terminator1 : Terminator
  vectorToQuaternion : Subsystem
  rate_setpoint : Outport
  prev_q : Outport  Port=2
  wires:
  pGain/1 -> Switch/3, Assignment/1, Selector/1
  Demux/3 -> Abs1/1
  att_sp_q/1 -> Cast To Single/1
  q/1 -> Quaternion Multiplication1/2, prev_q/1, MATLAB Function7/1(q), Quaternion Inverse1/1, Quaternion Inverse2/1
  Product4/1 -> Add/2
  Constant2/1 -> Subtract/2
  MATLAB Function1/1(v) -> vectorToQuaternion/2(dst)
  qDelta/1 -> Quaternion Multiplication/1
  Cast To Single/1 -> Normalize Vector/1
  Saturation2/1 -> Assignment2/2
  Switch1/1 -> Quaternion Multiplication3/1, Quaternion Inverse/1
  Normalize Vector/1 -> Quaternion Multiplication/2
  MATLAB Function3/1(v) -> Product4/1
  Quaternion Multiplication/1 -> Normalize Vector1/1
  Normalize Vector1/1 -> Quaternion Multiplication2/2, Switch1/1, MATLAB Function1/1(q)
  MATLAB Function7/1(v) -> vectorToQuaternion/1(src)
  Quaternion Inverse2/1 -> MATLAB Function3/1(q)
  vectorToQuaternion/1(quat) -> Quaternion Multiplication1/1, Demux/1
  Demux/1 -> Terminator/1
  MATLAB Function2/1(q_canonical) -> MATLAB Function4/1(q)
  Selector3/1 -> Acos/1
  Selector2/1 -> Saturation2/1
  Demux/2 -> Abs/1
  Demux/4 -> Terminator1/1
  Constant/1 -> Relational Operator/2
  Constant1/1 -> Subtract/1
  Quaternion Multiplication1/1 -> Switch1/3
  Abs/1 -> Relational Operator1/1
  Mux/1 -> Quaternion Multiplication3/2
  Relational Operator2/1 -> OR/2
  Abs1/1 -> Relational Operator2/1
  Subtract/1 -> Relational Operator1/2, Relational Operator2/2
  Relational Operator1/1 -> OR/1
  OR/1 -> Switch1/2
  Quaternion Inverse1/1 -> Quaternion Multiplication4/1
  Quaternion Inverse/1 -> Quaternion Multiplication2/1
  Selector/1 -> Divide/1
  Quaternion Multiplication2/1 -> MATLAB Function/1(q)
  Quaternion Multiplication4/1 -> MATLAB Function2/1(q)
  MATLAB Function/1(q_canonical) -> Assignment1/1, Selector1/1
  Selector1/1 -> Saturation1/1
  Cos/1 -> Mux/1
  Product1/1 -> Sin/1
  Saturation1/1 -> Assignment1/2
  Assignment1/1 -> Assignment2/1, Selector2/1
  Assignment2/1 -> Selector3/1, Selector4/1
  yawSpSetpoint/1 -> IsFinite/1, Product4/2
  Constant3/1 -> Mux/2
  yawWeight/1 -> Saturation/1
  Selector4/1 -> Asin/1
  Acos/1 -> Product/2
  Assignment/1 -> Switch/1
  Asin/1 -> Product1/2
  Saturation/1 -> Divide/2, Relational Operator/1, Product1/1, Product/1
  Product/1 -> Cos/1
  Divide/1 -> Assignment/2
  Relational Operator/1 -> Switch/2
  Sin/1 -> Mux/4
  Constant4/1 -> Mux/3
  Switch/1 -> Product3/2
  Quaternion Multiplication3/1 -> Quaternion Multiplication4/2
  Constant5/1 -> Product2/1
  MATLAB Function4/1(v) -> Product2/2
  Product2/1 -> Product3/1
  Product3/1 -> Switch2/3, Add/1
  Add/1 -> Switch2/1
  IsFinite/1 -> Switch2/2
  Switch2/1 -> Demux1/1
  Demux1/1 -> Saturation3/1
  Demux1/2 -> Saturation4/1
  Demux1/3 -> Saturation5/1
  Saturation3/1 -> Mux1/1
  Saturation4/1 -> Mux1/2
  Saturation5/1 -> Mux1/3
  Mux1/1 -> rate_setpoint/1
